simulink model "mas508_cw34_example2"  (R2021b)
settings: Solver=FixedStepDiscrete  StartTime=0.0  StopTime=10  FixedStep=1e-3  RelTol=1e-3
values from neighbouring files (symbols this model uses):
  b = 20    [mas508_cw34.m]    (also in mas508_lab2_exercise3_4.m = 0.06)
  F = 0    [mas508_cw34.m]
  k = 1000    [Lab6_example2_3.m]    (also in mas508_cw34.m = 1200; mas508_lab2_exercise2.m = 100; mas508_lab2_exercise3_4.m = 6)
  m = 11.2    [mas508_cw34.m]
undefined symbols (not defined in the file or in its folder): DiscIntNeverNeededParam
libraries: slrealtimeloglib x1
settings Model: Creator=rtavares  LastModifiedBy=faisala
settings SolverCC: ConcurrentTasks=on  AlgebraicLoopSolver=TrustRegion  PositivePriorityOrder=on
settings DataIOCC: ReturnWorkspaceOutputs=off
settings OptimizationCC: BlockReduction=off  OptimizeBlockIOStorage=off
settings DebuggingCC: TasksWithSamePriorityMsg=none  SFMachineParentedDataDiag=warning
settings HardwareCC: ProdBitPerLong=64  ProdLongLongMode=on  ProdHWDeviceType=Intel->x86-64 (Linux 64)
settings RTWCC: Description=Simulink Real-Time  SystemTargetFile=slrealtime.tlc  TemplateMakefile=slrealtime_default_tmf  Toolchain=Simulink Real-Time Toolchain  BuildConfiguration=Faster Runs  CodeExecutionProfiling=on  TargetLang=C++

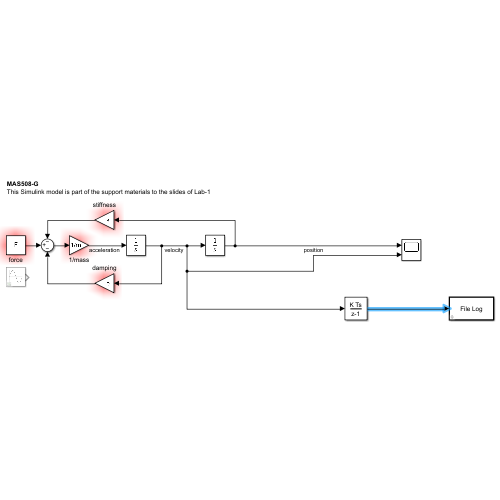
[thumbnail: Simulink's stored preview of the top-level diagram]
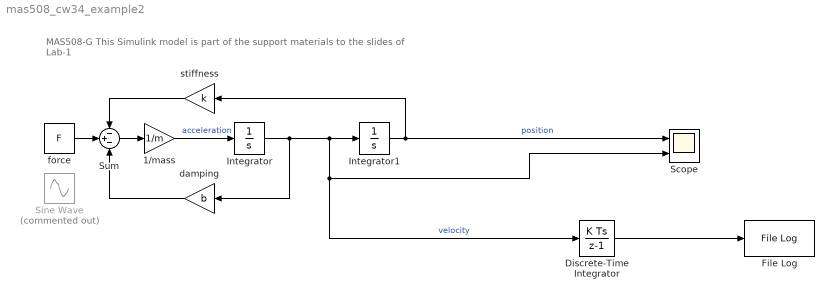
== system mas508_cw34_example2 ==
  note: MAS508-G
      | This Simulink model is part of the support materials to the slides of Lab-1
  1/mass : Gain  Gain=1/m
  Discrete-Time Integrator : DiscreteIntegrator  SampleTime=-1  ICPrevOutput=DiscIntNeverNeededParam  ICPrevScaledInput=DiscIntNeverNeededParam
  File Log : slrealtimeloglib/File Log  decimation=1
      settings: SourceProductBaseCode=XP
  Integrator : Integrator
  Integrator1 : Integrator  InitialCondition=1.5
  Scope : Scope  NumInputPorts=2
  Sine Wave : Sin  Commented=on  Amplitude=200  Frequency=2*pi*3  SampleTime=0
  Sum : Sum  Inputs=-+-
  damping : Gain  Gain=b
  force : Constant  Value=F
  stiffness : Gain  Gain=k
  wires:
  Integrator/1 -> damping/1, Discrete-Time Integrator/1, Scope/2, Integrator1/1  "velocity"
  Integrator1/1 -> stiffness/1, Scope/1  "position"
  1/mass/1 -> Integrator/1  "acceleration"
  Sum/1 -> 1/mass/1
  damping/1 -> Sum/3
  stiffness/1 -> Sum/1
  force/1 -> Sum/2
  Discrete-Time Integrator/1 -> File Log/1
